simulink model "MAN_ForceRAO"  (R2022a)
settings: Solver=ode4  StartTime=0.0  StopTime=1000  FixedStep=0.05  RelTol=1e-3  EnableMultiTasking=on
undefined symbols (not defined in the file): Hoerner, slcm, vessel
libraries: mssSimulink x6, simulink_extras x6
settings Model: Creator=Thor  LastModifiedBy=thor
settings SolverCC: AlgebraicLoopSolver=TrustRegion
settings DataIOCC: LimitDataPoints=on  SaveFormat=Array  SignalLoggingSaveFormat=ModelDataLogs  ReturnWorkspaceOutputs=off
settings OptimizationCC: ExpressionDepthLimit=2147483647  InitFltsAndDblsToZero=on  LifeSpan=inf
settings DebuggingCC: SaveWithParameterizedLinksMsg=none  UnderspecifiedInitializationDetection=Classic  MergeDetectMultiDrivingBlocksExec=none  SignalResolutionControl=TryResolveAllWithWarning  SolverPrmCheckMsg=warning  MultiTaskDSMMsg=warning  MultiTaskCondExecSysMsg=none  FcnCallInpInsideContextMsg=warning  UnconnectedInputMsg=warning  UnconnectedOutputMsg=warning  UnconnectedLineMsg=warning  StateNameClashWarn=warning  SFUnexpectedBacktrackingDiag=warning  SFNoUnconditionalDefaultTransitionDiag=warning  SFExecutionAtInitializationDiag=none  SFMachineParentedDataDiag=warning  ArithmeticOperatorsInVariantConditions=warning
settings HardwareCC: ProdBitPerPointer=32  ProdBitPerSizeT=32  ProdBitPerPtrDiffT=32  ProdLargestAtomicFloat=None  ProdIntDivRoundTo=Undefined  ProdEndianess=Unspecified  ProdWordSize=32  ProdHWDeviceType=32-bit Generic
settings ModelReferenceCC: PropagateSignalLabelsOutOfModel=off
settings SFSimCC: SimUseLocalCustomCode=off  CustomCodeUndefinedFunction=UseInterfaceOnly
settings RTWCC: RTWUseLocalCustomCode=off  DLArmComputeVersion=19.05
settings CodeAppCC: StateflowObjectComments=on
settings GRTTargetCC: TargetFcnLib=ansi_tfl_tmw.mat  TargetLangStandard=C89/C90 (ANSI)  CombineOutputUpdateFcns=off  GRTInterface=on
settings ConfigComp: CovMetricSettings=dw  CovSaveCumulativeToWorkspaceVar=on  CovSaveSingleToWorkspaceVar=on  CovExternalEMLEnable=off

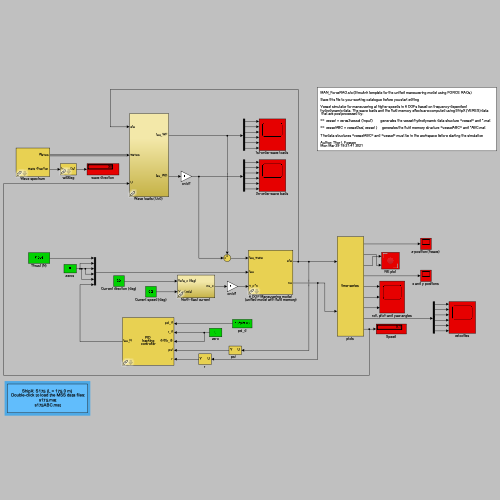
[thumbnail: Simulink's stored preview of the top-level diagram]
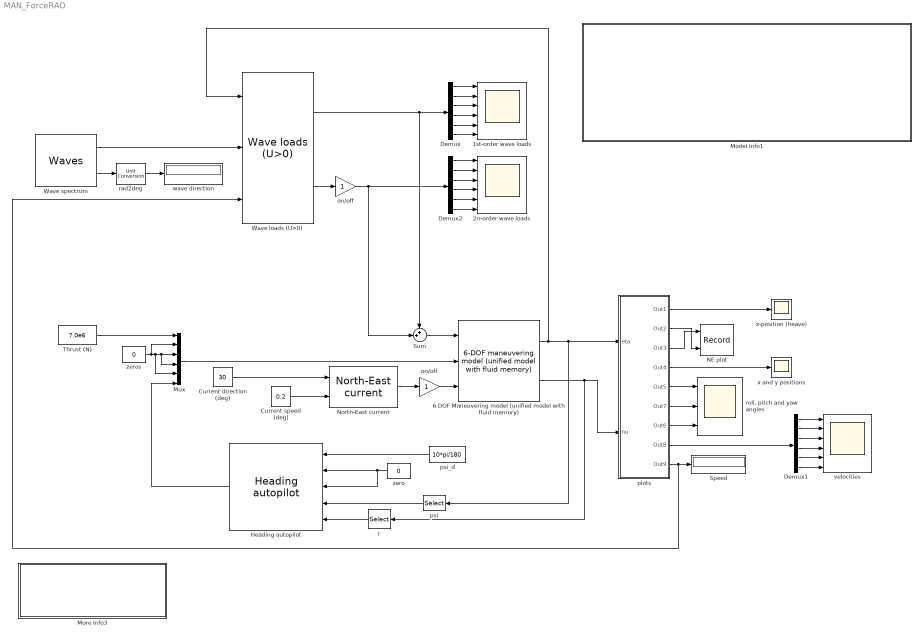
== system MAN_ForceRAO ==
  "1st-order wave loads " : Scope  NumInputPorts=6
  2n-order wave loads : Scope  NumInputPorts=6
  6 DOF Maneuvering model (unified model with fluid memory) : mssSimulink/Hydrodynamics/6-DOF maneuvering model  (unified model with fluid memory)  ABC=vesselABC  rho=1025  Axc=0.9*vessel.main.T*vessel.main.B  Ayc=0.9*vessel.main.T*vessel.main.Lpp  CX=1  CY_2D=Hoerner(vessel.main.B,vessel.main.T)
  Current direction (deg) : Constant  Value=30
  Current speed (deg) : Constant  Value=0.2
  Demux : Demux  Outputs=6
      settings: DisplayOption=none
  Demux1 : Demux  Outputs=6
      settings: DisplayOption=none
  Demux2 : Demux  Outputs=6
      settings: DisplayOption=none
  Heading autopilot : mssSimulink/Control/Autopilots/Heading autopilot  T_nomoto=10  K_nomoto=1/vessel.MRB(6,6)  Kp=1.0*vessel.MRB(6,6)  Td=10  Ti=50
  Model Info1 : Subsystem  LoadFcn=slcm LoadBlock;  InitFcn=slcm('UpdateAllCMBlocksInThisModelInit')  mask(CMBlock){InitialSaveTempField=, InitialBlockCM=None, BlockCM=None, Frame=on, SaveTempField=, DisplayStringWithTags=|, MaskDisplayString=MAN_ForceRAO.slx (Simulink template for the unified maneuvering model using FORCE RAOs)\n\nSave this file to your working catalogue before you start editing\n\nVessel simulator for maneuvering at higher speeds in 6 DOFs based on frequency-dependent\nhydrodynamic data. The wave loads and the fluid memory effects are computed using ShipX (VERES) data\n that are postprocessed by:\n\n>> vessel = veres2vessel ('input')        generates the vessel/hydrodynamic data structure <vessel> and *.mat \n\n>> vesselABC = vessel2ss( vessel )     generates the fluid memory structure <vesselABC> and *ABC.mat\n\nThe data structures <vesselABC> and <vessel> must be in the workspace before starting the simulation\n\nAuthor: Thor I. Fossen\nMon Mar 29 19:21:41 2021, HorizontalTextAlignment=Left, LeftAlignmentValue=0.02, SourceBlockDiagram=MAN_ForceRAO, TagMaxNumber=20, CMTag1=, CMTag2=, CMTag3=, CMTag4=, CMTag5=, CMTag6=, CMTag7=, CMTag8=, CMTag9=, CMTag10=, CMTag11=, CMTag12=, CMTag13=, CMTag14=, CMTag15=, CMTag16=, CMTag17=, CMTag18=, CMTag19=, CMTag20=}
      mask DisplayStringWithTags=|
      | MAN_ForceRAO.slx (Simulink template for the unified maneuvering model using FORCE RAOs)\n
      | Save this file to your working catalogue before you start editing\n
      | Vessel simulator for maneuvering at higher speeds in 6 DOFs based on frequency-dependent\nhydrodynamic data. The wave loads and the fluid memory effects are computed using ShipX (VERES) data\n that are postprocessed by:\n
      | >> vessel = veres2vessel ('input')        generates the vessel/hydrodynamic data structure <vessel> and *.mat
      |
      | >> vesselABC = vessel2ss( vessel )     generates the fluid memory structure <vesselABC> and *ABC.mat
      |
      | The data structures <vesselABC> and <vessel> must be in the workspace before starting the simulation
      |
      | Author: Thor I. Fossen
      | %<LastModificationDate>
      mask help: This block allows revision control information to be displayed within the model.
      settings: CopyFcn=slcm CopyBlock;  DeleteFcn=slcm Cancel;  PostSaveFcn=slcm('UpdateAllCMBlocksInThisModel')  NameChangeFcn=slcm Rename;  OpenFcn=slcm
      mask Display: text(str2num(LeftAlignmentValue), 0.5, MaskDisplayString, 'HorizontalAlignment', HorizontalTextAlignment)
  More Info3 : Subsystem
      settings: OpenFcn=load('s175'),load('s175ABC');disp('MSS S175 data set (L = 175.0 m) loaded')
      mask Display: disp('ShipX: S175 (L = 175.0 m)\n  Double-click to load the MSS data files:\n s175.mat\n s175ABC.mat')
  Mux : Mux  Inputs=6
  NE plot : Record  FileSettingsInternal="{\"entries\":[{\"content\":{\"excelSettings\":{\"content\":{},\"type\":\"Streamout.ExcelSettings\"}},\"type\":\"Streamout.FileSettingStorage\",\"uuid\":\"c64a618d-8b40-4725-8d6b-971e0d1a673d\"}],\"packageUris\":[\"http://schema.mathworks.com/mf0/streamout_blocks/R2020a\"],\"version\":\"1.0\"}"  Layout=[1 1]  SignalsInternal="{\"entries\":[{\"content\":{\"signals\":[{\"content\":{\"blockPath\":[\"MAN_ForceRAO/NE plot\"],\"channel\":[],\"dimensions\":[1],\"domain\":\"MAN_ForceRAO/NE plot\",\"lineColor\":\"#a2142f\",\"plots\":[1],\"port\":1,\"sid\":[\"\"],\"signalID\":1260,\"signalName\":\"plots:3\"},\"type\":\"RecordBlkView.Signal\",\"uuid\":\"cb114c13-d179-4bb3-ab4c-e5b4289d11a3\"},{\"content\":{\"blockPath\":[\"MAN_ForceRAO/NE plot\"],\"channel\":[],\"dimensions\":[1],\"domain\":\"MAN_ForceRAO/NE plot\",\"lineColor\":\"#139fff\",\"plots\":[1],\"port\":2,\"sid\":[\"\"],\"signalID\":1264,\"signalName\":\"plots:2\"},\"type\":\"RecordBlkView.Signal\",\"uuid\":\"19a96518-a1f5-4dc8-a269-b0be4ac5c1eb\"}]},\"type\":\"RecordBlkView.InputSignals\",\"uuid\":\"a8c6c26d-a06d-4548-9c48-70f15d8c45b1\"}],\"packageUris\":[\"http://schema.mathworks.com/mf0/streamout_blocks/R2020a\"],\"version\":\"1.0\"}"  VisualizationBindings="{\"xyplotplugin\":{\"info\":[{\"series\":[{\"bindingParametersList\":[{\"parameter\":\"X-Axis\",\"signalID\":1260,\"signalName\":\"plots:3\"},{\"parameter\":\"Y-Axis\",\"signalID\":1264,\"signalName\":\"plots:2\"}],\"seriesID\":26627}],\"subplotID\":1}]}}"  CompatibilityTag=XY  st=-1
  "North-East current " : mssSimulink/Environment/Current/North-East current  SystemSampleTime=-1  VariantActivationTime=update diagram  Latency=0  AutoFrameSizeCalculation=off
  Speed : Display
  Sum : Sum  Inputs=++|
  Thrust (N) : Constant  Value=7.0e6
  "Wave loads (U>0) " : mssSimulink/Hydrodynamics/Wave loads (U>0)  SystemSampleTime=-1  VariantActivationTime=update diagram  Latency=0  AutoFrameSizeCalculation=off
  Wave spectrum : mssSimulink/Environment/Waves/Waves  spectrum_type=ITTC  disp_flag=off  plot_spectrum=off  plot_realization=off  hs=3  omega_peak=-1  psi_mean=30*pi/180  gamma=-1  spread=2  depth=inf  nfreq=20  ndir=10  energylim=0.005  freq_cutoff=3  dir_cutoff=0  rand_seed=0  rand_freq=on  rand_dir=on  Zeta_a=0  Omega=0  Phase=0  Wavenum=0  Psi=0
  on/off : Gain
  "on/off " : Gain
  plots : Subsystem
      mask Display: disp('time-series')
  "psi   " : Selector  InputPortWidth=6  IndexOptions=Index vector (dialog)  Indices=[6]  OutputSizes=1
  psi_d : Constant  Value=10*pi/180
  r : Selector  InputPortWidth=6  IndexOptions=Index vector (dialog)  Indices=[6]  OutputSizes=1
  rad2deg : mssSimulink/Utilities/Math Operations/Unit Conversion  in=rad2deg
  "roll, pitch and yaw angles" : Scope  NumInputPorts=3
  velocities : Scope  NumInputPorts=6
  wave direction : Display
  x and y positions : Scope
  z-position (heave) : Scope
  zero : Constant  Value=0
  zeros : Constant  Value=0
  wires:
  plots/3(Out3) -> NE plot/1
  plots/2(Out2) -> NE plot/2
  plots/4(Out4) -> x and y positions/1
  Demux/1 -> "1st-order wave loads "/1
  Demux/2 -> "1st-order wave loads "/2
  Demux/3 -> "1st-order wave loads "/3
  Demux/4 -> "1st-order wave loads "/4
  Demux/5 -> "1st-order wave loads "/5
  Demux/6 -> "1st-order wave loads "/6
  plots/5(Out5) -> "roll, pitch and yaw angles"/1
  plots/6(Out7) -> "roll, pitch and yaw angles"/2
  plots/7(Out6) -> "roll, pitch and yaw angles"/3
  plots/1(Out1) -> z-position (heave)/1
  "Wave loads (U>0) "/2 -> on/off/1
  Wave spectrum/1 -> "Wave loads (U>0) "/2
  Demux1/1 -> velocities/1
  Demux1/2 -> velocities/2
  Demux1/3 -> velocities/3
  Demux1/4 -> velocities/4
  Demux1/5 -> velocities/5
  Demux1/6 -> velocities/6
  plots/8(Out8) -> Demux1/1
  Wave spectrum/2 -> rad2deg/1
  rad2deg/1 -> wave direction/1
  Demux2/1 -> 2n-order wave loads/1
  Demux2/2 -> 2n-order wave loads/2
  Demux2/3 -> 2n-order wave loads/3
  Demux2/4 -> 2n-order wave loads/4
  Demux2/5 -> 2n-order wave loads/5
  Demux2/6 -> 2n-order wave loads/6
  Sum/1 -> 6 DOF Maneuvering model (unified model with fluid memory)/1
  "Wave loads (U>0) "/1 -> Demux/1, Sum/1
  on/off/1 -> Sum/2, Demux2/1
  "North-East current "/1 -> "on/off "/1
  "on/off "/1 -> 6 DOF Maneuvering model (unified model with fluid memory)/3
  Current speed (deg)/1 -> "North-East current "/2
  Current direction (deg)/1 -> "North-East current "/1
  plots/9(Out9) -> Speed/1, "Wave loads (U>0) "/3
  Thrust (N)/1 -> Mux/1
  "psi   "/1 -> Heading autopilot/4
  zero/1 -> Heading autopilot/2, Heading autopilot/3
  psi_d/1 -> Heading autopilot/1
  Heading autopilot/1 -> Mux/6
  zeros/1 -> Mux/2, Mux/3, Mux/4, Mux/5
  Mux/1 -> 6 DOF Maneuvering model (unified model with fluid memory)/2
  r/1 -> Heading autopilot/5
  6 DOF Maneuvering model (unified model with fluid memory)/1 -> plots/1(eta), "psi   "/1, "Wave loads (U>0) "/1
  6 DOF Maneuvering model (unified model with fluid memory)/2 -> plots/2(nu), r/1

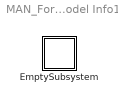
== system MAN_ForceRAO/Model Info1 ==
  EmptySubsystem : Subsystem

== system MAN_ForceRAO/More Info3 ==

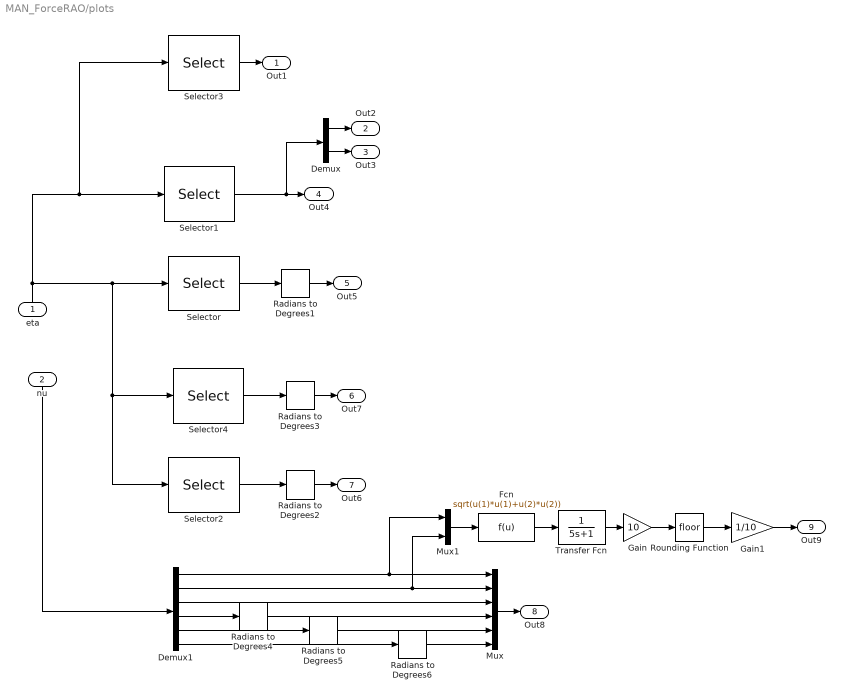
== system MAN_ForceRAO/plots ==
  eta : Inport
  nu : Inport  Port=2
  Demux : Demux  Outputs=2
      settings: DisplayOption=none
  Demux1 : Demux  Outputs=6
      settings: DisplayOption=none
  Fcn : Fcn  Expr=sqrt(u(1)*u(1)+u(2)*u(2))
  Gain : Gain  Gain=10
  Gain1 : Gain  Gain=1/10
  Mux : Mux  Inputs=6
  Mux1 : Mux  Inputs=2
  Radians to Degrees{1..6} (6 alike) : simulink_extras/Transformations/Radians to Degrees
  Rounding Function : Rounding
  Selector : Selector  InputPortWidth=6  IndexOptions=Index vector (dialog)  Indices=[4 ]  OutputSizes=1
  Selector1 : Selector  InputPortWidth=6  IndexOptions=Index vector (dialog)  Indices=[1 2]  OutputSizes=1
  Selector2 : Selector  InputPortWidth=6  IndexOptions=Index vector (dialog)  Indices=[6]  OutputSizes=1
  Selector3 : Selector  InputPortWidth=6  IndexOptions=Index vector (dialog)  Indices=[3]  OutputSizes=1
  Selector4 : Selector  InputPortWidth=6  IndexOptions=Index vector (dialog)  Indices=[5]  OutputSizes=1
  Transfer Fcn : TransferFcn  Denominator=[5 1]
  Out1 : Outport
  Out2 : Outport  Port=2
  Out3 : Outport  Port=3
  Out4 : Outport  Port=4
  Out5 : Outport  Port=5
  Out7 : Outport  Port=6
  Out6 : Outport  Port=7
  Out8 : Outport  Port=8
  Out9 : Outport  Port=9
  wires:
  eta/1 -> Selector3/1, Selector1/1, Selector/1, Selector2/1, Selector4/1
  Selector/1 -> Radians to Degrees1/1
  Selector1/1 -> Demux/1, Out4/1
  Selector2/1 -> Radians to Degrees2/1
  Selector3/1 -> Out1/1
  Demux/1 -> Out2/1
  Demux/2 -> Out3/1
  Radians to Degrees1/1 -> Out5/1
  Radians to Degrees2/1 -> Out6/1
  Selector4/1 -> Radians to Degrees3/1
  Radians to Degrees3/1 -> Out7/1
  nu/1 -> Demux1/1
  Demux1/1 -> Mux/1, Mux1/1
  Demux1/2 -> Mux/2, Mux1/2
  Demux1/3 -> Mux/3
  Demux1/4 -> Radians to Degrees4/1
  Demux1/5 -> Radians to Degrees5/1
  Demux1/6 -> Radians to Degrees6/1
  Radians to Degrees6/1 -> Mux/6
  Radians to Degrees5/1 -> Mux/5
  Radians to Degrees4/1 -> Mux/4
  Mux/1 -> Out8/1
  Fcn/1 -> Transfer Fcn/1
  Mux1/1 -> Fcn/1
  Rounding Function/1 -> Gain1/1
  Gain/1 -> Rounding Function/1
  Gain1/1 -> Out9/1
  Transfer Fcn/1 -> Gain/1

== system MAN_ForceRAO/Model Info1/EmptySubsystem ==
